simulink model "archifinale"  (R2016a)
settings: Solver=VariableStepAuto  StartTime=0.0  StopTime=90  RelTol=1e-3
undefined symbols (not defined in the file): A, B, b, C, Continuous, D, F, K, MIL, Nbar, R_kalman, Time, Ts, W
libraries: aerolibfltsims x2, aerolibwind2 x1, mpclib x1, aerolibtransform2 x1, ctrlSharedLib x1
settings Model: Creator=User  LastModifiedBy=User

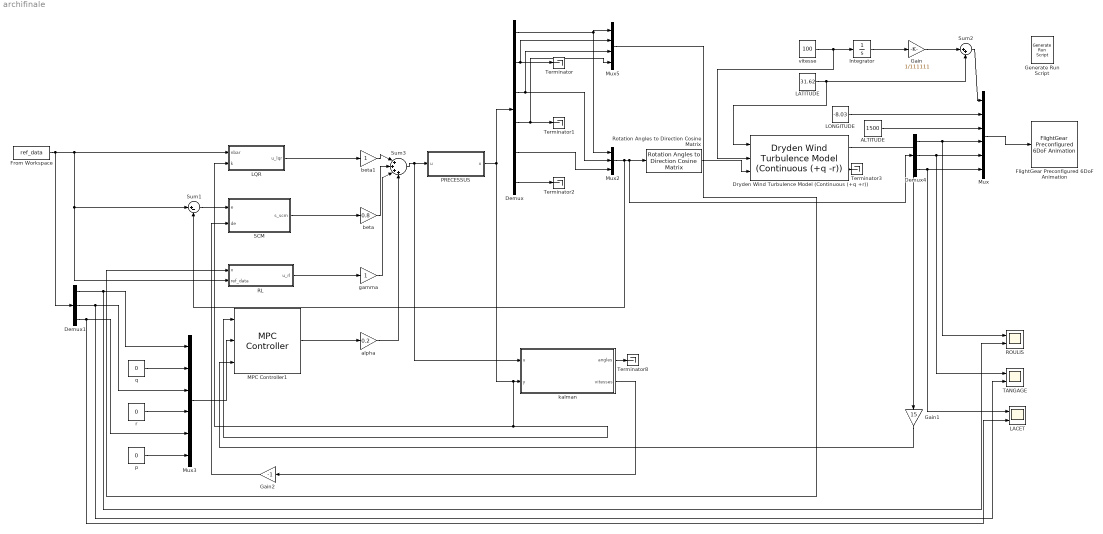
== system archifinale ==
  ALTITUDE : Constant  Value=1500
  Demux : Demux  Outputs=6
  Demux1 : Demux  Outputs=3
  Demux4 : Demux  Outputs=3
  Dryden Wind Turbulence Model (Continuous (+q +r)) : aerolibwind2/Dryden Wind Turbulence Model  (Continuous (+q -r))  units=Metric (MKS)  spec=MIL-F-8785C  model=Continuous Dryden (+q +r)  W20=5  Wdeg=0  TurbProb=10^-1  L_high=533.4  Wingspan=10  ts=0.01  Seed=[23341 23342 23343 23344]  T_on=on
  FlightGear Preconfigured 6DoF Animation : aerolibfltsims/FlightGear Preconfigured 6DoF Animation  xFlightGearVersion=v3.4  DestinationIpAddress=127.0.0.1  DestinationPort=5502  SampleTime=1/30
  From Workspace : FromWorkspace  VariableName=ref_data  OutDataTypeStr=double  SampleTime=Ts
  Gain : Gain  Gain=1/111111
  Gain1 : Gain  Gain=15
  Gain2 : Gain  Gain=-1
  Generate Run Script : aerolibfltsims/Generate Run Script  OutputFileName=runfg.bat  FlightGearBaseDirectory=C:\Program Files\FlightGear  GeometryModelName=HL20  DestinationPort=5502  OriginAddress=127.0.0.1  OriginPort=5505  LocalAddress=127.0.0.1  AirportId=KSFO  RunwayId=10L  InitialAltitude=7224  InitialHeading=113  OffsetDistance=4.72  OffsetAzimuth=0  GenerateFile=off  Architecture=Default  dataFlow=Send
  Integrator : Integrator
  LACET : Scope  NumInputPorts=2
  LATITUDE : Constant  Value=31.62
  LONGITUDE : Constant  Value=-8.03
  LQR : Subsystem
  MPC Controller1 : mpclib/MPC Controller  SCDEnableBlockLinearizationSpecification=on  mpcobj=mpcobj  is_multiple=0  enable_value=0  return_u0=off  ref_from_ws=off  ref_signal_name=[]  ref_preview=off  md_from_ws=off  md_signal_name=[]  md_preview=off  from_project=off  project_file=MPCtask.mat  md_inport=on  mv_inport=off  cost_outport=off  return_sequence=off  return_qpstatus=off  return_state=off  state_inport=off  lims_inport=off  ywt_inport=off  is_designfromscratch=0  uwt_inport=off  duwt_inport=off  rhoeps_inport=off  uref_inport=off  n_ts=0.05  n_mv=4  n_md=3  n_ud=0  n_mo=6  n_uo=0  BlockDataType=double  SampleTimeInherited=off  switch_inport=off
  Mux : Mux  Inputs=6
  Mux2 : Mux  Inputs=3
  Mux3 : Mux  Inputs=6
  Mux5 : Mux
  PRECESSUS : Subsystem
  "RL " : Subsystem
  ROULIS : Scope  NumInputPorts=2
  Rotation Angles to Direction Cosine Matrix : aerolibtransform2/Rotation Angles to Direction Cosine Matrix  rotationOrder=ZYX
  SCM : Subsystem
  Sum1 : Sum  Inputs=|+-
  Sum2 : Sum  Inputs=|++
  Sum3 : Sum  Inputs=|++++
  TANGAGE : Scope  NumInputPorts=2
  Terminator{,1..3,8} (5 alike) : Terminator
  alpha : Gain  Gain=0.2
  beta : Gain  Gain=0.8
  beta1 : Gain
  gamma : Gain
  kalman : Subsystem
  p : Constant  Value=0
  q : Constant  Value=0
  r : Constant  Value=0
  vitesse : Constant  Value=100
  wires:
  Mux/1 -> FlightGear Preconfigured 6DoF Animation/1
  ALTITUDE/1 -> Mux/3
  LONGITUDE/1 -> Mux/2
  vitesse/1 -> Dryden Wind Turbulence Model (Continuous (+q +r))/2, Integrator/1
  Integrator/1 -> Gain/1
  Gain/1 -> Sum2/1
  LATITUDE/1 -> Sum2/2, Dryden Wind Turbulence Model (Continuous (+q +r))/1
  Sum2/1 -> Mux/1
  PRECESSUS/1(x) -> MPC Controller1/1, LQR/2("k "), kalman/2(y), Demux/1
  Dryden Wind Turbulence Model (Continuous (+q +r))/1 -> Gain1/1
  Mux2/1 -> Rotation Angles to Direction Cosine Matrix/1, Demux4/1, Sum1/2
  Rotation Angles to Direction Cosine Matrix/1 -> Dryden Wind Turbulence Model (Continuous (+q +r))/3
  Demux/2 -> Terminator/1, Mux5/2
  Demux/4 -> Mux5/4, Terminator1/1
  Demux/6 -> Terminator2/1
  Dryden Wind Turbulence Model (Continuous (+q +r))/2 -> Terminator3/1
  Mux3/1 -> MPC Controller1/2
  Demux1/3 -> LACET/2, Mux3/5
  Demux1/1 -> Mux3/1, ROULIS/2
  Demux1/2 -> TANGAGE/2, Mux3/3
  q/1 -> Mux3/2
  kalman/2(vitesses) -> Gain2/1
  Sum1/1 -> SCM/1(e)
  p/1 -> Mux3/6
  r/1 -> Mux3/4
  LQR/1(u_lqr) -> beta1/1
  Sum3/1 -> kalman/1(u), PRECESSUS/1(u)
  SCM/1(s_scm) -> beta/1
  beta1/1 -> Sum3/1
  From Workspace/1 -> Demux1/1, LQR/1(nbar), "RL "/2(ref_data), Sum1/1
  beta/1 -> Sum3/2
  "RL "/1(u_rl) -> gamma/1
  gamma/1 -> Sum3/3
  MPC Controller1/1 -> alpha/1
  alpha/1 -> Sum3/4
  Gain2/1 -> SCM/2(de)
  Demux/1 -> Mux5/1, Mux2/1
  Demux/3 -> Mux2/2, Mux5/3
  Demux/5 -> Mux2/3
  Mux5/1 -> "RL "/1(x)
  Gain1/1 -> MPC Controller1/3
  Demux4/1 -> ROULIS/1, Mux/4
  Demux4/2 -> TANGAGE/1, Mux/5
  Demux4/3 -> LACET/1, Mux/6
  kalman/1("angles ") -> Terminator8/1

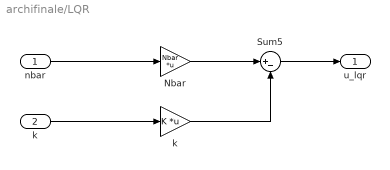
== system archifinale/LQR ==
  nbar : Inport
  "k " : Inport  Port=2
  Nbar : Gain  Gain=Nbar  Multiplication=Matrix(K*u)
  Sum5 : Sum  Inputs=|+-
  k : Gain  Gain=K  Multiplication=Matrix(K*u)
  u_lqr : Outport
  wires:
  Nbar/1 -> Sum5/1
  k/1 -> Sum5/2
  Sum5/1 -> u_lqr/1
  "k "/1 -> k/1
  nbar/1 -> Nbar/1

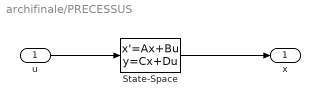
== system archifinale/PRECESSUS ==
  u : Inport
  State-Space : StateSpace  A=A  B=B  C=C  D=D  X0=0
  x : Outport
  wires:
  u/1 -> State-Space/1
  State-Space/1 -> x/1

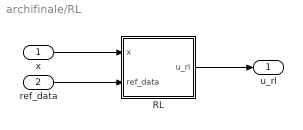
== system archifinale/RL  ==
  x : Inport
  ref_data : Inport  Port=2
  RL : MATLAB Function  TreatAsAtomicUnit=on
  u_rl : Outport
  wires:
  RL/1(u_rl) -> u_rl/1
  x/1 -> RL/1(x)
  ref_data/1 -> RL/2(ref_data)

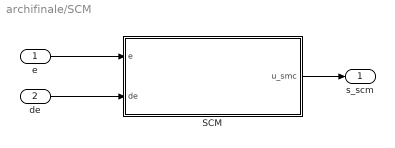
== system archifinale/SCM ==
  e : Inport
  de : Inport  Port=2
  "SCM " : MATLAB Function  TreatAsAtomicUnit=on
  s_scm : Outport
  wires:
  "SCM "/1(u_smc) -> s_scm/1
  e/1 -> "SCM "/1(e)
  de/1 -> "SCM "/2(de)

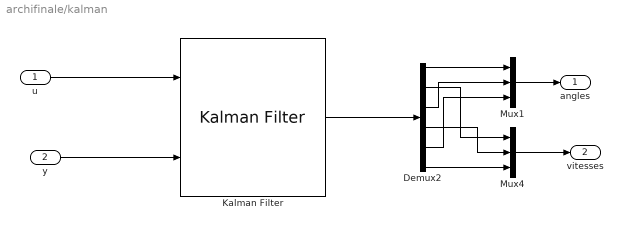
== system archifinale/kalman ==
  u : Inport
  y : Inport  Port=2
  Demux2 : Demux  Outputs=6
  Kalman Filter : ctrlSharedLib/Kalman Filter  TimeDomain=Continuous-Time  UseCurrentEstimator=on  ModelSource=Individual A, B, C, D matrices  ModelSourceVariable=kalman_est  A=A  B=B  C=C  D=D  NumberOfStates=1  NumberOfInputs=1  NumberOfOutputs=1  InitialEstimateSource=Dialog  X0=0  P0=10  UseK=off  UseGH=off  NumberOfProcessNoiseInputs=1  G=1  TimeInvariantG=on  H=0  TimeInvariantH=on  Q=Q_kalman  TimeInvariantQ=on  R=R_kalman  TimeInvariantR=on  N=0  TimeInvariantN=on  AddInputPort=on  AddEnablePort=off  ExternalReset=none  OutputEstimatedY=off  OutputP=off  Ts=-1
  Mux1 : Mux  Inputs=3
  Mux4 : Mux  Inputs=3
  "angles " : Outport
  vitesses : Outport  Port=2
  wires:
  y/1 -> Kalman Filter/2
  Kalman Filter/1 -> Demux2/1
  Demux2/1 -> Mux1/1
  Demux2/3 -> Mux1/2
  Demux2/5 -> Mux1/3
  Demux2/6 -> Mux4/3
  Demux2/4 -> Mux4/2
  Demux2/2 -> Mux4/1
  u/1 -> Kalman Filter/1
  Mux1/1 -> "angles "/1
  Mux4/1 -> vitesses/1

== matlab function archifinale/RL /RL ==
  data: x input double size=4; ref_data input double size=3; W parameter double size=2 4; b parameter double size=2 1; u_rl output double size=4
function u_rl = ai_corrector(x, ref_data, W, b)
    u_rl = zeros(4, 1);
    
    roll_ref  = ref_data(1);
    pitch_ref = ref_data(2);
    
    err_roll  = x(1) - roll_ref;
    err_pitch = x(3) - pitch_ref;
    
    nn_in = [err_roll; x(2); err_pitch; x(4)];
    
    correction = W * nn_in + b;
    
    % GAINS DIFFERENTS : roll faible, pitch fort
    u_rl(1) = correction(1) * 0.05;   % roll : très doux (déjà bon)
    u_rl(2) = correction(2) * 0.5;   % pitch : plus fort (à améliorer)
end

== matlab function archifinale/SCM/SCM  ==
  data: e input double size=3; u_smc output double size=4; de input
function u_smc = fcn(e, de)
    % ============================================================
    % SMC ADDITIF - Sortie 4x1 [da, de, dr, dthrottle]
    % ============================================================
    
    % Paramètres
    lambda = [4.0; 6.0; 2.5];   % 3x1
    k = [1.5; 2.5; 1.0];       % 3x1
    phi = 0.15;                 % scalaire
    
    % Surface de glissement (3x1)
    s = de + lambda .* e;       % e et de doivent être 3x1
    
    % Saturation lisse (3x1)
    sat = s ./ (abs(s) + phi);
    
    % Commande de commutation (3x1)
    u_sw = -k .* sat;
    
    % ============================================================
    % MAPPING VERS 4 ENTRÉES (OBLIGATOIRE)
    % ============================================================
    u_smc = zeros(4,1);         % <-- 4x1, pas 6x1 !
    u_smc(1) = u_sw(1);         % aileron  (roulis)
    u_smc(2) = u_sw(2) + (0.05 * e(2));         % elevator (tangage)
    u_smc(3) = u_sw(3);         % rudder   (lacet)
    u_smc(4) = 0;               % throttle = 0 (LQR gère)
    
    % Saturation
    u_smc(1) = max(min(u_smc(1), 0.436), -0.436);
    u_smc(2) = max(min(u_smc(2), 0.17), -0.17);
    u_smc(3) = max(min(u_smc(3), 0.524), -0.524);
    u_smc(4) = max(min(u_smc(4), 1.0), -1.0);   % throttle ±100%
    
end
